simulink model "GaN_Clamp_Wide_Range_Analog_State"  (R2022b)
settings: Solver=ode15s  StartTime=0.0  StopTime=3e-6  MaxStep=5e-10  RelTol=1e-7  AbsTol=1e-9
model workspace (MAT data in the model file):
  btb_wide_150V_negative = [0 1e-10 2e-10 3e-10 4e-10 5e-10 6e-10 7e-10 8e-10 9e-10 1e-09 1.1e-09 ... (60002 elements, 30001x2)]
  btb_wide_150V_positive = [0 1e-10 2e-10 3e-10 4e-10 5e-10 6e-10 7e-10 8e-10 9e-10 1e-09 1.1e-09 ... (60002 elements, 30001x2)]
  btb_wide_400V_negative = [0 1e-10 2e-10 3e-10 4e-10 5e-10 6e-10 7e-10 8e-10 9e-10 1e-09 1.1e-09 ... (60002 elements, 30001x2)]
  btb_wide_400V_positive = [0 1e-10 2e-10 3e-10 4e-10 5e-10 6e-10 7e-10 8e-10 9e-10 1e-09 1.1e-09 ... (60002 elements, 30001x2)]
  btb_wide_50V_negative = [0 1e-10 2e-10 3e-10 4e-10 5e-10 6e-10 7e-10 8e-10 9e-10 1e-09 1.1e-09 ... (60002 elements, 30001x2)]
  btb_wide_50V_positive = [0 1e-10 2e-10 3e-10 4e-10 5e-10 6e-10 7e-10 8e-10 9e-10 1e-09 1.1e-09 ... (60002 elements, 30001x2)]
  dv_wide_150V_negative = [0 1e-10 2e-10 3e-10 4e-10 5e-10 6e-10 7e-10 8e-10 9e-10 1e-09 1.1e-09 ... (60002 elements, 30001x2)]
  dv_wide_150V_positive = [0 1e-10 2e-10 3e-10 4e-10 5e-10 6e-10 7e-10 8e-10 9e-10 1e-09 1.1e-09 ... (60002 elements, 30001x2)]
  dv_wide_400V_negative = [0 1e-10 2e-10 3e-10 4e-10 5e-10 6e-10 7e-10 8e-10 9e-10 1e-09 1.1e-09 ... (60002 elements, 30001x2)]
  dv_wide_400V_positive = [0 1e-10 2e-10 3e-10 4e-10 5e-10 6e-10 7e-10 8e-10 9e-10 1e-09 1.1e-09 ... (60002 elements, 30001x2)]
  dv_wide_50V_negative = [0 1e-10 2e-10 3e-10 4e-10 5e-10 6e-10 7e-10 8e-10 9e-10 1e-09 1.1e-09 ... (60002 elements, 30001x2)]
  dv_wide_50V_positive = [0 1e-10 2e-10 3e-10 4e-10 5e-10 6e-10 7e-10 8e-10 9e-10 1e-09 1.1e-09 ... (60002 elements, 30001x2)]
  gb_wide_150V_negative = [0 1e-10 2e-10 3e-10 4e-10 5e-10 6e-10 7e-10 8e-10 9e-10 1e-09 1.1e-09 ... (60002 elements, 30001x2)]
  gb_wide_150V_positive = [0 1e-10 2e-10 3e-10 4e-10 5e-10 6e-10 7e-10 8e-10 9e-10 1e-09 1.1e-09 ... (60002 elements, 30001x2)]
  gb_wide_400V_negative = [0 1e-10 2e-10 3e-10 4e-10 5e-10 6e-10 7e-10 8e-10 9e-10 1e-09 1.1e-09 ... (60002 elements, 30001x2)]
  gb_wide_400V_positive = [0 1e-10 2e-10 3e-10 4e-10 5e-10 6e-10 7e-10 8e-10 9e-10 1e-09 1.1e-09 ... (60002 elements, 30001x2)]
  gb_wide_50V_negative = [0 1e-10 2e-10 3e-10 4e-10 5e-10 6e-10 7e-10 8e-10 9e-10 1e-09 1.1e-09 ... (60002 elements, 30001x2)]
  gb_wide_50V_positive = [0 1e-10 2e-10 3e-10 4e-10 5e-10 6e-10 7e-10 8e-10 9e-10 1e-09 1.1e-09 ... (60002 elements, 30001x2)]
  v_wide_150V_negative = [0 1e-10 2e-10 3e-10 4e-10 5e-10 6e-10 7e-10 8e-10 9e-10 1e-09 1.1e-09 ... (60002 elements, 30001x2)]
  v_wide_150V_positive = [0 1e-10 2e-10 3e-10 4e-10 5e-10 6e-10 7e-10 8e-10 9e-10 1e-09 1.1e-09 ... (60002 elements, 30001x2)]
  v_wide_400V_negative = [0 1e-10 2e-10 3e-10 4e-10 5e-10 6e-10 7e-10 8e-10 9e-10 1e-09 1.1e-09 ... (60002 elements, 30001x2)]
  v_wide_400V_positive = [0 1e-10 2e-10 3e-10 4e-10 5e-10 6e-10 7e-10 8e-10 9e-10 1e-09 1.1e-09 ... (60002 elements, 30001x2)]
  v_wide_50V_negative = [0 1e-10 2e-10 3e-10 4e-10 5e-10 6e-10 7e-10 8e-10 9e-10 1e-09 1.1e-09 ... (60002 elements, 30001x2)]
  v_wide_50V_positive = [0 1e-10 2e-10 3e-10 4e-10 5e-10 6e-10 7e-10 8e-10 9e-10 1e-09 1.1e-09 ... (60002 elements, 30001x2)]
settings Model: Creator=Greatlovers  LastModifiedBy=Greatlovers

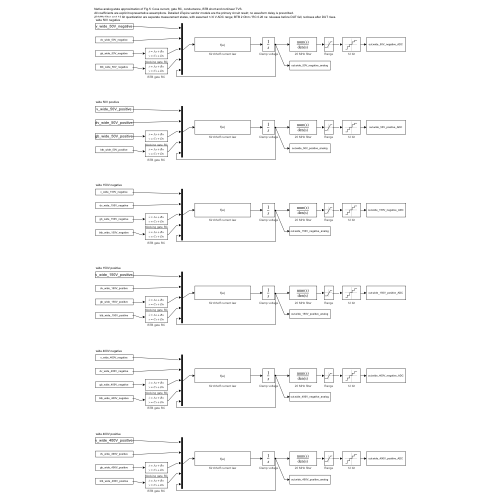
[thumbnail: Simulink's stored preview of the top-level diagram]
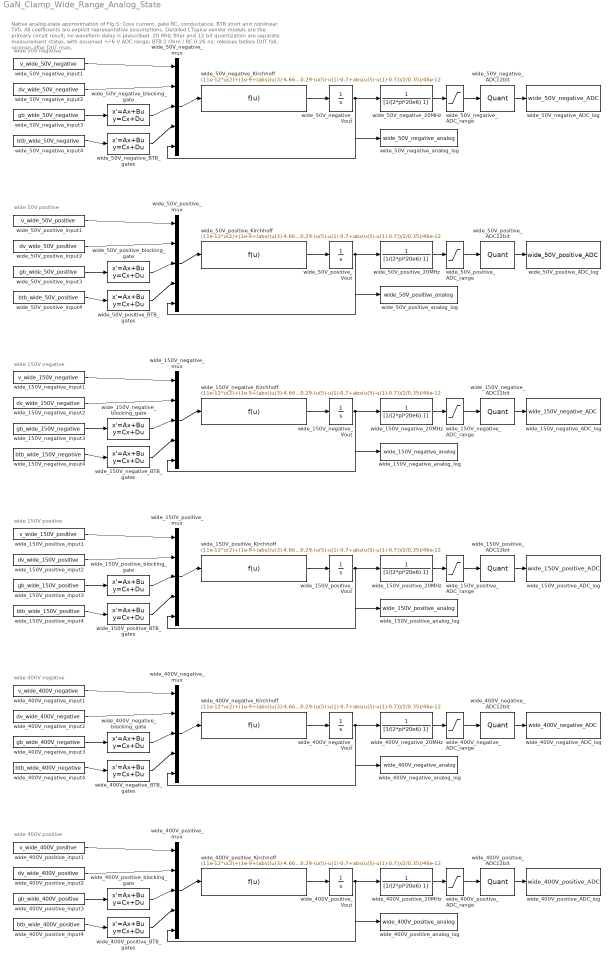
== system GaN_Clamp_Wide_Range_Analog_State ==
  note: wide 50V negative
  note: wide 50V positive
  note: wide 150V negative
  note: wide 150V positive
  note: wide 400V negative
  note: wide 400V positive
  note: Native analog-state approximation of Fig.5: Coss current, gate RC, conductance, BTB short and nonlinear TVS.
      | All coefficients are explicit representative assumptions. Detailed LTspice vendor models are the primary circuit result; no waveform delay is prescribed.
      | 20 MHz filter and 12 bit quantization are separate measurement states, with assumed +/-6 V ADC range; BTB 2 Ohm / RC 0.26 ns: releases before DUT fall, recloses after DUT rises.
  wide_150V_negative_20MHz : TransferFcn  Numerator=1  Denominator=[1/(2*pi*20e6) 1]
      settings: AttributesFormatString=20 MHz filter
  wide_150V_negative_ADC12bit : Quantizer  QuantizationInterval=0.0029296875
      settings: AttributesFormatString=12 bit
  wide_150V_negative_ADC_log : ToWorkspace  VariableName=wide_150V_negative_ADC  SaveFormat=Timeseries  SampleTime=-1
  wide_150V_negative_ADC_range : Saturate  UpperLimit=6  LowerLimit=-6
      settings: AttributesFormatString=Range
  wide_150V_negative_BTB_gates : StateSpace  A=-1/0.26e-9  B=1/0.26e-9  D=0  InitialCondition=4.5
      settings: AttributesFormatString=BTB gate RC
  wide_150V_negative_Kirchhoff : Fcn  Expr=(11e-12*u(2)+(1e-9+(abs((u(3)-4.662)/5.338)-abs((u(3)-4.662)/5.338-1)+1)/2/11)*(u(1)-u(5))-(abs((u(4)-0.6118)/3.8882)-abs((u(4)-0.6118)/3.8882-1)+1)/2/0.122*u(5)-u(5)/1e6-((u(5)-8+abs(u(5)-8))/2-(-u(5)-8+abs(-u(5)-8))/2)/0.29-(u(5)-u(1)-0.7+abs(u(5)-u(1)-0.7))/2/0.35)/46e-12
      settings: AttributesFormatString=Kirchhoff current law
  wide_150V_negative_Vout : Integrator
      settings: AttributesFormatString=Clamp voltage
  wide_150V_negative_analog_log : ToWorkspace  VariableName=wide_150V_negative_analog  SaveFormat=Timeseries  SampleTime=-1
  wide_150V_negative_blocking_gate : StateSpace  A=-1/1.88e-9  B=1/1.88e-9  D=0  InitialCondition=0
      settings: AttributesFormatString=Blocking gate RC
  wide_150V_negative_input1 : FromWorkspace  VariableName=v_wide_150V_negative
  wide_150V_negative_input2 : FromWorkspace  VariableName=dv_wide_150V_negative
  wide_150V_negative_input3 : FromWorkspace  VariableName=gb_wide_150V_negative
  wide_150V_negative_input4 : FromWorkspace  VariableName=btb_wide_150V_negative
  wide_150V_negative_mux : Mux  Inputs=5
  wide_150V_positive_20MHz : TransferFcn  Numerator=1  Denominator=[1/(2*pi*20e6) 1]
      settings: AttributesFormatString=20 MHz filter
  wide_150V_positive_ADC12bit : Quantizer  QuantizationInterval=0.0029296875
      settings: AttributesFormatString=12 bit
  wide_150V_positive_ADC_log : ToWorkspace  VariableName=wide_150V_positive_ADC  SaveFormat=Timeseries  SampleTime=-1
  wide_150V_positive_ADC_range : Saturate  UpperLimit=6  LowerLimit=-6
      settings: AttributesFormatString=Range
  wide_150V_positive_BTB_gates : StateSpace  A=-1/0.26e-9  B=1/0.26e-9  D=0  InitialCondition=4.5
      settings: AttributesFormatString=BTB gate RC
  wide_150V_positive_Kirchhoff : Fcn  Expr=(11e-12*u(2)+(1e-9+(abs((u(3)-4.662)/5.338)-abs((u(3)-4.662)/5.338-1)+1)/2/11)*(u(1)-u(5))-(abs((u(4)-0.6118)/3.8882)-abs((u(4)-0.6118)/3.8882-1)+1)/2/0.122*u(5)-u(5)/1e6-((u(5)-8+abs(u(5)-8))/2-(-u(5)-8+abs(-u(5)-8))/2)/0.29-(u(5)-u(1)-0.7+abs(u(5)-u(1)-0.7))/2/0.35)/46e-12
      settings: AttributesFormatString=Kirchhoff current law
  wide_150V_positive_Vout : Integrator
      settings: AttributesFormatString=Clamp voltage
  wide_150V_positive_analog_log : ToWorkspace  VariableName=wide_150V_positive_analog  SaveFormat=Timeseries  SampleTime=-1
  wide_150V_positive_blocking_gate : StateSpace  A=-1/1.88e-9  B=1/1.88e-9  D=0  InitialCondition=0
      settings: AttributesFormatString=Blocking gate RC
  wide_150V_positive_input1 : FromWorkspace  VariableName=v_wide_150V_positive
  wide_150V_positive_input2 : FromWorkspace  VariableName=dv_wide_150V_positive
  wide_150V_positive_input3 : FromWorkspace  VariableName=gb_wide_150V_positive
  wide_150V_positive_input4 : FromWorkspace  VariableName=btb_wide_150V_positive
  wide_150V_positive_mux : Mux  Inputs=5
  wide_400V_negative_20MHz : TransferFcn  Numerator=1  Denominator=[1/(2*pi*20e6) 1]
      settings: AttributesFormatString=20 MHz filter
  wide_400V_negative_ADC12bit : Quantizer  QuantizationInterval=0.0029296875
      settings: AttributesFormatString=12 bit
  wide_400V_negative_ADC_log : ToWorkspace  VariableName=wide_400V_negative_ADC  SaveFormat=Timeseries  SampleTime=-1
  wide_400V_negative_ADC_range : Saturate  UpperLimit=6  LowerLimit=-6
      settings: AttributesFormatString=Range
  wide_400V_negative_BTB_gates : StateSpace  A=-1/0.26e-9  B=1/0.26e-9  D=0  InitialCondition=4.5
      settings: AttributesFormatString=BTB gate RC
  wide_400V_negative_Kirchhoff : Fcn  Expr=(11e-12*u(2)+(1e-9+(abs((u(3)-4.662)/5.338)-abs((u(3)-4.662)/5.338-1)+1)/2/11)*(u(1)-u(5))-(abs((u(4)-0.6118)/3.8882)-abs((u(4)-0.6118)/3.8882-1)+1)/2/0.122*u(5)-u(5)/1e6-((u(5)-8+abs(u(5)-8))/2-(-u(5)-8+abs(-u(5)-8))/2)/0.29-(u(5)-u(1)-0.7+abs(u(5)-u(1)-0.7))/2/0.35)/46e-12
      settings: AttributesFormatString=Kirchhoff current law
  wide_400V_negative_Vout : Integrator
      settings: AttributesFormatString=Clamp voltage
  wide_400V_negative_analog_log : ToWorkspace  VariableName=wide_400V_negative_analog  SaveFormat=Timeseries  SampleTime=-1
  wide_400V_negative_blocking_gate : StateSpace  A=-1/1.88e-9  B=1/1.88e-9  D=0  InitialCondition=0
      settings: AttributesFormatString=Blocking gate RC
  wide_400V_negative_input1 : FromWorkspace  VariableName=v_wide_400V_negative
  wide_400V_negative_input2 : FromWorkspace  VariableName=dv_wide_400V_negative
  wide_400V_negative_input3 : FromWorkspace  VariableName=gb_wide_400V_negative
  wide_400V_negative_input4 : FromWorkspace  VariableName=btb_wide_400V_negative
  wide_400V_negative_mux : Mux  Inputs=5
  wide_400V_positive_20MHz : TransferFcn  Numerator=1  Denominator=[1/(2*pi*20e6) 1]
      settings: AttributesFormatString=20 MHz filter
  wide_400V_positive_ADC12bit : Quantizer  QuantizationInterval=0.0029296875
      settings: AttributesFormatString=12 bit
  wide_400V_positive_ADC_log : ToWorkspace  VariableName=wide_400V_positive_ADC  SaveFormat=Timeseries  SampleTime=-1
  wide_400V_positive_ADC_range : Saturate  UpperLimit=6  LowerLimit=-6
      settings: AttributesFormatString=Range
  wide_400V_positive_BTB_gates : StateSpace  A=-1/0.26e-9  B=1/0.26e-9  D=0  InitialCondition=4.5
      settings: AttributesFormatString=BTB gate RC
  wide_400V_positive_Kirchhoff : Fcn  Expr=(11e-12*u(2)+(1e-9+(abs((u(3)-4.662)/5.338)-abs((u(3)-4.662)/5.338-1)+1)/2/11)*(u(1)-u(5))-(abs((u(4)-0.6118)/3.8882)-abs((u(4)-0.6118)/3.8882-1)+1)/2/0.122*u(5)-u(5)/1e6-((u(5)-8+abs(u(5)-8))/2-(-u(5)-8+abs(-u(5)-8))/2)/0.29-(u(5)-u(1)-0.7+abs(u(5)-u(1)-0.7))/2/0.35)/46e-12
      settings: AttributesFormatString=Kirchhoff current law
  wide_400V_positive_Vout : Integrator
      settings: AttributesFormatString=Clamp voltage
  wide_400V_positive_analog_log : ToWorkspace  VariableName=wide_400V_positive_analog  SaveFormat=Timeseries  SampleTime=-1
  wide_400V_positive_blocking_gate : StateSpace  A=-1/1.88e-9  B=1/1.88e-9  D=0  InitialCondition=0
      settings: AttributesFormatString=Blocking gate RC
  wide_400V_positive_input1 : FromWorkspace  VariableName=v_wide_400V_positive
  wide_400V_positive_input2 : FromWorkspace  VariableName=dv_wide_400V_positive
  wide_400V_positive_input3 : FromWorkspace  VariableName=gb_wide_400V_positive
  wide_400V_positive_input4 : FromWorkspace  VariableName=btb_wide_400V_positive
  wide_400V_positive_mux : Mux  Inputs=5
  wide_50V_negative_20MHz : TransferFcn  Numerator=1  Denominator=[1/(2*pi*20e6) 1]
      settings: AttributesFormatString=20 MHz filter
  wide_50V_negative_ADC12bit : Quantizer  QuantizationInterval=0.0029296875
      settings: AttributesFormatString=12 bit
  wide_50V_negative_ADC_log : ToWorkspace  VariableName=wide_50V_negative_ADC  SaveFormat=Timeseries  SampleTime=-1
  wide_50V_negative_ADC_range : Saturate  UpperLimit=6  LowerLimit=-6
      settings: AttributesFormatString=Range
  wide_50V_negative_BTB_gates : StateSpace  A=-1/0.26e-9  B=1/0.26e-9  D=0  InitialCondition=4.5
      settings: AttributesFormatString=BTB gate RC
  wide_50V_negative_Kirchhoff : Fcn  Expr=(11e-12*u(2)+(1e-9+(abs((u(3)-4.662)/5.338)-abs((u(3)-4.662)/5.338-1)+1)/2/11)*(u(1)-u(5))-(abs((u(4)-0.6118)/3.8882)-abs((u(4)-0.6118)/3.8882-1)+1)/2/0.122*u(5)-u(5)/1e6-((u(5)-8+abs(u(5)-8))/2-(-u(5)-8+abs(-u(5)-8))/2)/0.29-(u(5)-u(1)-0.7+abs(u(5)-u(1)-0.7))/2/0.35)/46e-12
      settings: AttributesFormatString=Kirchhoff current law
  wide_50V_negative_Vout : Integrator
      settings: AttributesFormatString=Clamp voltage
  wide_50V_negative_analog_log : ToWorkspace  VariableName=wide_50V_negative_analog  SaveFormat=Timeseries  SampleTime=-1
  wide_50V_negative_blocking_gate : StateSpace  A=-1/1.88e-9  B=1/1.88e-9  D=0  InitialCondition=0
      settings: AttributesFormatString=Blocking gate RC
  wide_50V_negative_input1 : FromWorkspace  VariableName=v_wide_50V_negative
  wide_50V_negative_input2 : FromWorkspace  VariableName=dv_wide_50V_negative
  wide_50V_negative_input3 : FromWorkspace  VariableName=gb_wide_50V_negative
  wide_50V_negative_input4 : FromWorkspace  VariableName=btb_wide_50V_negative
  wide_50V_negative_mux : Mux  Inputs=5
  wide_50V_positive_20MHz : TransferFcn  Numerator=1  Denominator=[1/(2*pi*20e6) 1]
      settings: AttributesFormatString=20 MHz filter
  wide_50V_positive_ADC12bit : Quantizer  QuantizationInterval=0.0029296875
      settings: AttributesFormatString=12 bit
  wide_50V_positive_ADC_log : ToWorkspace  VariableName=wide_50V_positive_ADC  SaveFormat=Timeseries  SampleTime=-1
  wide_50V_positive_ADC_range : Saturate  UpperLimit=6  LowerLimit=-6
      settings: AttributesFormatString=Range
  wide_50V_positive_BTB_gates : StateSpace  A=-1/0.26e-9  B=1/0.26e-9  D=0  InitialCondition=4.5
      settings: AttributesFormatString=BTB gate RC
  wide_50V_positive_Kirchhoff : Fcn  Expr=(11e-12*u(2)+(1e-9+(abs((u(3)-4.662)/5.338)-abs((u(3)-4.662)/5.338-1)+1)/2/11)*(u(1)-u(5))-(abs((u(4)-0.6118)/3.8882)-abs((u(4)-0.6118)/3.8882-1)+1)/2/0.122*u(5)-u(5)/1e6-((u(5)-8+abs(u(5)-8))/2-(-u(5)-8+abs(-u(5)-8))/2)/0.29-(u(5)-u(1)-0.7+abs(u(5)-u(1)-0.7))/2/0.35)/46e-12
      settings: AttributesFormatString=Kirchhoff current law
  wide_50V_positive_Vout : Integrator
      settings: AttributesFormatString=Clamp voltage
  wide_50V_positive_analog_log : ToWorkspace  VariableName=wide_50V_positive_analog  SaveFormat=Timeseries  SampleTime=-1
  wide_50V_positive_blocking_gate : StateSpace  A=-1/1.88e-9  B=1/1.88e-9  D=0  InitialCondition=0
      settings: AttributesFormatString=Blocking gate RC
  wide_50V_positive_input1 : FromWorkspace  VariableName=v_wide_50V_positive
  wide_50V_positive_input2 : FromWorkspace  VariableName=dv_wide_50V_positive
  wide_50V_positive_input3 : FromWorkspace  VariableName=gb_wide_50V_positive
  wide_50V_positive_input4 : FromWorkspace  VariableName=btb_wide_50V_positive
  wide_50V_positive_mux : Mux  Inputs=5
  wires:
  wide_50V_negative_input1/1 -> wide_50V_negative_mux/1
  wide_50V_negative_input2/1 -> wide_50V_negative_mux/2
  wide_50V_negative_input3/1 -> wide_50V_negative_blocking_gate/1
  wide_50V_negative_input4/1 -> wide_50V_negative_BTB_gates/1
  wide_50V_negative_blocking_gate/1 -> wide_50V_negative_mux/3
  wide_50V_negative_BTB_gates/1 -> wide_50V_negative_mux/4
  wide_50V_negative_mux/1 -> wide_50V_negative_Kirchhoff/1
  wide_50V_negative_Kirchhoff/1 -> wide_50V_negative_Vout/1
  wide_50V_negative_Vout/1 -> wide_50V_negative_mux/5, wide_50V_negative_20MHz/1, wide_50V_negative_analog_log/1
  wide_50V_negative_20MHz/1 -> wide_50V_negative_ADC_range/1
  wide_50V_negative_ADC_range/1 -> wide_50V_negative_ADC12bit/1
  wide_50V_negative_ADC12bit/1 -> wide_50V_negative_ADC_log/1
  wide_50V_positive_input1/1 -> wide_50V_positive_mux/1
  wide_50V_positive_input2/1 -> wide_50V_positive_mux/2
  wide_50V_positive_input3/1 -> wide_50V_positive_blocking_gate/1
  wide_50V_positive_input4/1 -> wide_50V_positive_BTB_gates/1
  wide_50V_positive_blocking_gate/1 -> wide_50V_positive_mux/3
  wide_50V_positive_BTB_gates/1 -> wide_50V_positive_mux/4
  wide_50V_positive_mux/1 -> wide_50V_positive_Kirchhoff/1
  wide_50V_positive_Kirchhoff/1 -> wide_50V_positive_Vout/1
  wide_50V_positive_Vout/1 -> wide_50V_positive_mux/5, wide_50V_positive_20MHz/1, wide_50V_positive_analog_log/1
  wide_50V_positive_20MHz/1 -> wide_50V_positive_ADC_range/1
  wide_50V_positive_ADC_range/1 -> wide_50V_positive_ADC12bit/1
  wide_50V_positive_ADC12bit/1 -> wide_50V_positive_ADC_log/1
  wide_150V_negative_input1/1 -> wide_150V_negative_mux/1
  wide_150V_negative_input2/1 -> wide_150V_negative_mux/2
  wide_150V_negative_input3/1 -> wide_150V_negative_blocking_gate/1
  wide_150V_negative_input4/1 -> wide_150V_negative_BTB_gates/1
  wide_150V_negative_blocking_gate/1 -> wide_150V_negative_mux/3
  wide_150V_negative_BTB_gates/1 -> wide_150V_negative_mux/4
  wide_150V_negative_mux/1 -> wide_150V_negative_Kirchhoff/1
  wide_150V_negative_Kirchhoff/1 -> wide_150V_negative_Vout/1
  wide_150V_negative_Vout/1 -> wide_150V_negative_mux/5, wide_150V_negative_20MHz/1, wide_150V_negative_analog_log/1
  wide_150V_negative_20MHz/1 -> wide_150V_negative_ADC_range/1
  wide_150V_negative_ADC_range/1 -> wide_150V_negative_ADC12bit/1
  wide_150V_negative_ADC12bit/1 -> wide_150V_negative_ADC_log/1
  wide_150V_positive_input1/1 -> wide_150V_positive_mux/1
  wide_150V_positive_input2/1 -> wide_150V_positive_mux/2
  wide_150V_positive_input3/1 -> wide_150V_positive_blocking_gate/1
  wide_150V_positive_input4/1 -> wide_150V_positive_BTB_gates/1
  wide_150V_positive_blocking_gate/1 -> wide_150V_positive_mux/3
  wide_150V_positive_BTB_gates/1 -> wide_150V_positive_mux/4
  wide_150V_positive_mux/1 -> wide_150V_positive_Kirchhoff/1
  wide_150V_positive_Kirchhoff/1 -> wide_150V_positive_Vout/1
  wide_150V_positive_Vout/1 -> wide_150V_positive_mux/5, wide_150V_positive_20MHz/1, wide_150V_positive_analog_log/1
  wide_150V_positive_20MHz/1 -> wide_150V_positive_ADC_range/1
  wide_150V_positive_ADC_range/1 -> wide_150V_positive_ADC12bit/1
  wide_150V_positive_ADC12bit/1 -> wide_150V_positive_ADC_log/1
  wide_400V_negative_input1/1 -> wide_400V_negative_mux/1
  wide_400V_negative_input2/1 -> wide_400V_negative_mux/2
  wide_400V_negative_input3/1 -> wide_400V_negative_blocking_gate/1
  wide_400V_negative_input4/1 -> wide_400V_negative_BTB_gates/1
  wide_400V_negative_blocking_gate/1 -> wide_400V_negative_mux/3
  wide_400V_negative_BTB_gates/1 -> wide_400V_negative_mux/4
  wide_400V_negative_mux/1 -> wide_400V_negative_Kirchhoff/1
  wide_400V_negative_Kirchhoff/1 -> wide_400V_negative_Vout/1
  wide_400V_negative_Vout/1 -> wide_400V_negative_mux/5, wide_400V_negative_20MHz/1, wide_400V_negative_analog_log/1
  wide_400V_negative_20MHz/1 -> wide_400V_negative_ADC_range/1
  wide_400V_negative_ADC_range/1 -> wide_400V_negative_ADC12bit/1
  wide_400V_negative_ADC12bit/1 -> wide_400V_negative_ADC_log/1
  wide_400V_positive_input1/1 -> wide_400V_positive_mux/1
  wide_400V_positive_input2/1 -> wide_400V_positive_mux/2
  wide_400V_positive_input3/1 -> wide_400V_positive_blocking_gate/1
  wide_400V_positive_input4/1 -> wide_400V_positive_BTB_gates/1
  wide_400V_positive_blocking_gate/1 -> wide_400V_positive_mux/3
  wide_400V_positive_BTB_gates/1 -> wide_400V_positive_mux/4
  wide_400V_positive_mux/1 -> wide_400V_positive_Kirchhoff/1
  wide_400V_positive_Kirchhoff/1 -> wide_400V_positive_Vout/1
  wide_400V_positive_Vout/1 -> wide_400V_positive_mux/5, wide_400V_positive_20MHz/1, wide_400V_positive_analog_log/1
  wide_400V_positive_20MHz/1 -> wide_400V_positive_ADC_range/1
  wide_400V_positive_ADC_range/1 -> wide_400V_positive_ADC12bit/1
  wide_400V_positive_ADC12bit/1 -> wide_400V_positive_ADC_log/1
